simulink model "Controller_torque_cbf_m22"  (R2022b)
settings: Solver=ode4  StartTime=0.0  StopTime=Inf  FixedStep=1e-3  RelTol=1e-3
values from neighbouring files (symbols this model uses):
  Dn = 20 * ones(7,1)    [init_torque_cbf.m]
  H_0_cy = H_0_pr * H_pr_cy    [init_torque_cbf.m]
  H_home = getTransform(Franka_robot, q_home, 'panda_link8', 'panda_link0')    [init_torque_cbf.m]
  Kn = 0 * ones(7,1)    [init_torque_cbf.m]
  q_home = q_init    [init_torque_cbf.m]
  q_init = [0 0  0  -(2/4)*pi  0  pi/2  -pi/4]'    [init_torque_cbf.m]
undefined symbols (not defined in the file or in its folder): cbf_torque_params, DiscIntNeverNeededParam, Fext_mag, T_final, X, Y, Z
libraries: sm_lib x162, nesl_utility x44, matrix_library x3, Robotics_lib x1
(part 12 of 12)

== matlab function Controller_torque_cbf_m22/task space controller/MATLAB Function2 ==
  data: H_IT input; x_c output size=1; v_c output size=1; V_tilde input; lambda_mat input; n_hp input; m_c output size=1; xTableHight input; eef_height input
function [x_c, v_c, m_c] = fcn(H_IT, V_tilde, lambda_mat, n_hp, xTableHight, eef_height)

auxMat = zeros(4,4);
auxMat(3,4) = -xTableHight;

H = H_IT*[eye(3), [0;0;eef_height];zeros(1,3),1] + auxMat;

x_c = transpose(n_hp)*[H(1:3,4);zeros(3,1)];

v_c = transpose(n_hp)*V_tilde;




lambda_inv = lambda_mat\eye(6);
lambda_inv = (lambda_inv + transpose(lambda_inv))./2;

tmp3 = transpose(n_hp)*lambda_inv*n_hp;
m_c = tmp3\eye(1);


end
